simulink model "Lag"  (R2022a)
settings: Solver=VariableStepAuto  StartTime=0.0  StopTime=10.0  RelTol=1e-3
settings Model: Creator=user  LastModifiedBy=user

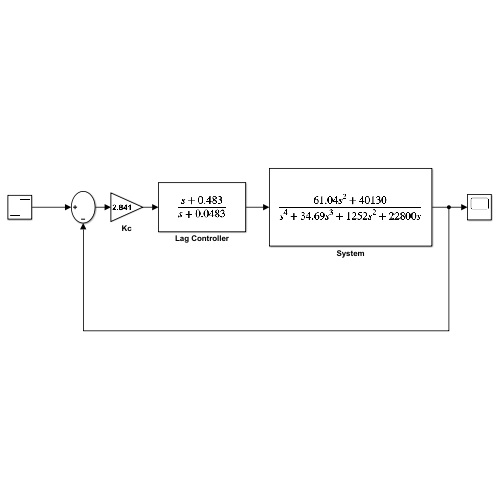
[thumbnail: Simulink's stored preview of the top-level diagram]
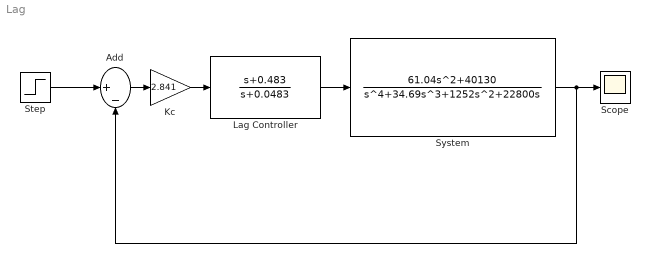
== system Lag ==
  Add : Sum  Inputs=|+-
  Kc : Gain  Gain=2.841
  Lag Controller : TransferFcn  Numerator=[1 0.483]  Denominator=[1 0.0483]
  Scope : Scope
  Step : Step  Time=0  SampleTime=0
  System : TransferFcn  Numerator="[61.04 0  40130  ]"  Denominator=[1 34.69 1252 22800 0]
  wires:
  Lag Controller/1 -> System/1
  Step/1 -> Add/1
  System/1 -> Scope/1, Add/2
  Add/1 -> Kc/1
  Kc/1 -> Lag Controller/1
